simulink model "protect_check"  (R2023a)
settings: configuration reference "config" (kept outside this file)
model workspace (MAT data in the model file):
  timer_s = Simulink.Signal
  timer_s.Description = '时间计数器 s'
  timer_s.DataType = 'single'
  timer_s.Dimensions = -1
  timer_s.DimensionsMode = 'auto'
  timer_s.Complexity = 'auto'
  timer_s.SampleTime = -1
  timer_s.SamplingMode = 'auto'
  timer_s.InitialValue = '0'
settings Model: DataDictionary=model_config.sldd  Creator=huangcheng  LastModifiedBy=Administrator
settings ConfigSetRef: SourceName=config

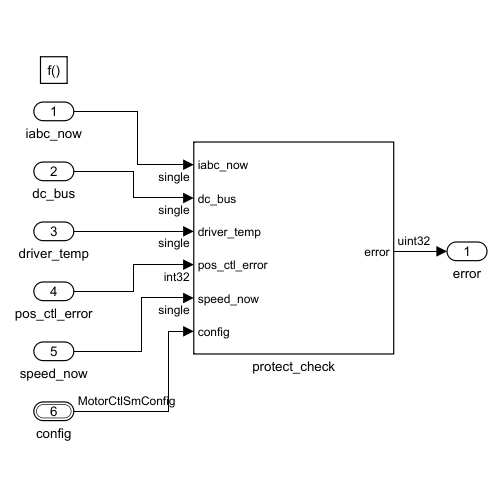
[thumbnail: Simulink's stored preview of the top-level diagram]
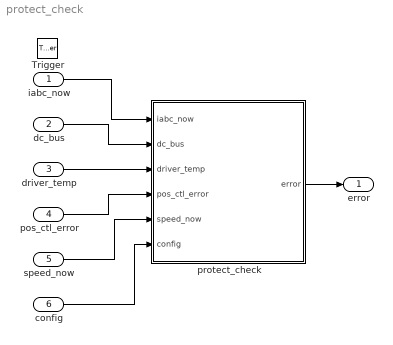
== system protect_check ==
  iabc_now : Inport
  dc_bus : Inport  Port=2
  driver_temp : Inport  Port=3
  pos_ctl_error : Inport  Port=4
  speed_now : Inport  Port=5
  config : Inport  Port=6  OutDataTypeStr=Bus: MotorCtlSmConfig  BusOutputAsStruct=on
  Trigger : TriggerPort  TriggerType=function-call  VariantControl=(inherit)  PortDimensions=1
  protect_check : Subsystem
  error : Outport
  wires:
  config/1 -> protect_check/6(config)
  speed_now/1 -> protect_check/5(speed_now)
  pos_ctl_error/1 -> protect_check/4(pos_ctl_error)
  driver_temp/1 -> protect_check/3(driver_temp)
  dc_bus/1 -> protect_check/2(dc_bus)
  iabc_now/1 -> protect_check/1(iabc_now)
  protect_check/1(error) -> error/1

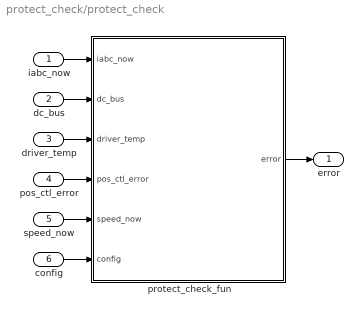
== system protect_check/protect_check ==
  iabc_now : Inport  OutDataTypeStr=single  PortDimensions=3
  dc_bus : Inport  Port=2  OutDataTypeStr=single
  driver_temp : Inport  Port=3  OutDataTypeStr=single
  pos_ctl_error : Inport  Port=4  OutDataTypeStr=int32
  speed_now : Inport  Port=5  OutDataTypeStr=single
  config : Inport  Port=6  OutDataTypeStr=Bus: MotorCtlSmConfig
  protect_check_fun : MATLAB Function  TreatAsAtomicUnit=on
  error : Outport  OutDataTypeStr=uint32
  wires:
  iabc_now/1 -> protect_check_fun/1(iabc_now)
  dc_bus/1 -> protect_check_fun/2(dc_bus)
  driver_temp/1 -> protect_check_fun/3(driver_temp)
  pos_ctl_error/1 -> protect_check_fun/4(pos_ctl_error)
  speed_now/1 -> protect_check_fun/5(speed_now)
  config/1 -> protect_check_fun/6(config)
  protect_check_fun/1(error) -> error/1

== matlab function protect_check/protect_check_fun ==
  data: iabc_now input; error output; dc_bus input; driver_temp input; pos_ctl_error input; speed_now input; config input
function error = protect_check(iabc_now, dc_bus, driver_temp, pos_ctl_error, speed_now, config)
 
% config.error_enable  保护可以根据配置关闭 开启



%电压保护
if dc_bus < config.under_voltage_protection_V && bitget(config.error_enable, 1) == 1
    error = uint32(1);
    return;
end

if dc_bus > config.over_voltage_protection_V  && bitget(config.error_enable, 2) == 1 
    error = uint32(2);
    return;
end


%过流保护
if iabc_now(1) > config.over_current_protection_A  && bitget(config.error_enable, 7) == 1  
    error = uint32(7);
    return;
end
if iabc_now(1) < -config.over_current_protection_A && bitget(config.error_enable, 7) == 1   
    error = uint32(7);
    return;
end

if iabc_now(2) > config.over_current_protection_A && bitget(config.error_enable, 7) == 1   
    error = uint32(7);
    return;
end
if iabc_now(2) < -config.over_current_protection_A && bitget(config.error_enable, 7) == 1   
    error = uint32(7);
    return;
end

if iabc_now(3) > config.over_current_protection_A && bitget(config.error_enable, 7) == 1   
    error = uint32(7);
    return;
end
if iabc_now(3) < -config.over_current_protection_A && bitget(config.error_enable, 7) == 1   
    error = uint32(7);
    return;
end

%温度保护
if driver_temp < config.under_temperature_protection_d && bitget(config.error_enable, 4) == 1   
    error = uint32(4);
    return;
end
if driver_temp > config.over_temperature_protection_d && bitget(config.error_enable, 5) == 1   
    error = uint32(5);
    return;
end

%过速保护
if speed_now > config.over_speed_protection_rad_s && bitget(config.error_enable, 3) == 1    
    error = uint32(3);
    return;
end
if speed_now < -config.over_speed_protection_rad_s && bitget(config.error_enable, 3) == 1    
    error = uint32(3);
    return;
end


%位置跟随误差保护
if config.mode == 3 || config.mode == 4   %位置模式下才会生效位置误差保护

    if pos_ctl_error > config.position_following_error_protection && bitget(config.error_enable, 6) == 1    
        error = uint32(6);
        return;
    end
    if pos_ctl_error < -config.position_following_error_protection && bitget(config.error_enable, 6) == 1    
        error = uint32(6);
        return;
    end

end


error = uint32(0);
